simulink model "Pay_load"  (R2025a)
settings: Solver=ode4  StartTime=0.0  StopTime=1  FixedStep=0.001  RelTol=1e-3
values from neighbouring files (symbols this model uses):
  angle1_init = [0;0;0.3]    [param.m]
  angle2_init = [0;0;0.3]    [param.m]
  angle3_init = [0;0;0.3]    [param.m]
  angle4_init = [0;0;0.3]    [param.m]
  joint_matrix = [r1; r2; r3; r4]    [param.m]
  m1 = 1    [param.m]
  m2 = 1    [param.m]
  m3 = 1    [param.m]
  m4 = 1    [param.m]
  mL = 2    [param.m]
  P = block.DialogPrm(1).Data    [Load_dynamic.m]    (also in param.m = struct())
  p1_init = pL_init + RL_init*r1 - l1*e1    [param.m]
  p2_init = pL_init + RL_init*r2 - l2*e2    [param.m]
  p3_init = pL_init + RL_init*r3 - l3*e3    [param.m]
  p4_init = pL_init + RL_init*r4 - l4*e4    [param.m]
  r1 = [ 0.25; -0.20; -0.45]    [param.m]
  r2 = [-0.50; -0.40; -0.15]    [param.m]
  r3 = [-0.50;  0.40;  0.15]    [param.m]
  r4 = [ 0.50;  0.40;  0.00]    [param.m]
  xL_init = [pL_init; vL_init; angle_L_init; omega_L_init]    [param.m]
(part 1 of 3)
settings Model: Creator=huy01  LastModifiedBy=huy01

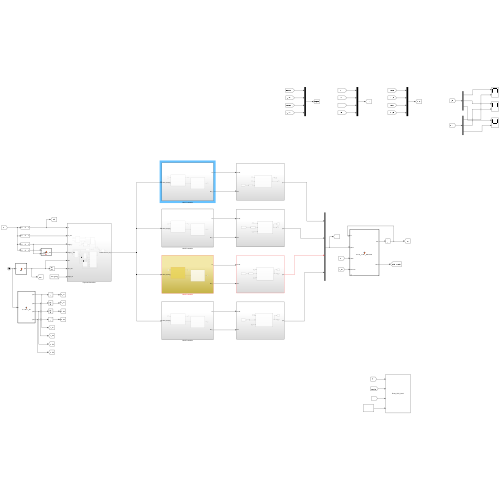
[thumbnail: Simulink's stored preview of the top-level diagram]
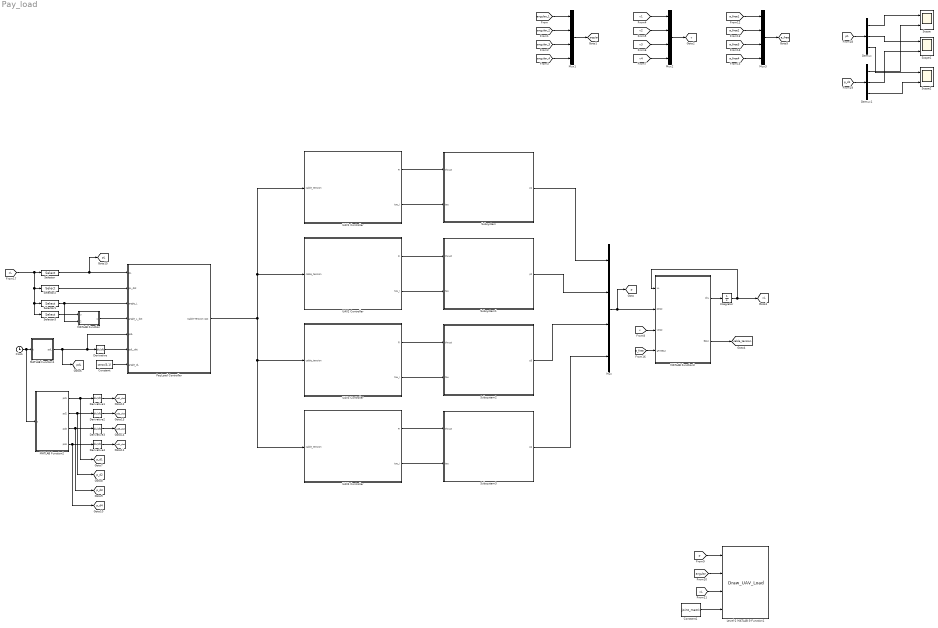
== system Pay_load ==
  Clock : Clock
  Constant : Constant  Value=zeros(3,1)
  Constant1 : Constant  Value=joint_matrix
  Demux : Demux  Outputs=3
  Demux1 : Demux  Outputs=3
  Derivative{,1..4} (5 alike) : Derivative
  Integrator : Integrator  InitialCondition=xL_init
  Level-2 MATLAB S-Function1 : M-S-Function  FunctionName=Draw_UAV_Load
  MATLAB Function : MATLAB Function  TreatAsAtomicUnit=on
  MATLAB Function1 : MATLAB Function  TreatAsAtomicUnit=on
  MATLAB Function2 : MATLAB Function  TreatAsAtomicUnit=on
  MATLAB Function3 : MATLAB Function  TreatAsAtomicUnit=on  mask{P=P}
      mask prompts: P "Struct param"
  Mux{,1..3} (4 alike) : Mux
  PayLoad Controller : Subsystem
  Scope : Scope  NumInputPorts=2
      settings: ActiveDisplayYMinimum=-0.075646367743774853  ActiveDisplayYMaximum=0.68476273102431728  DataLoggingVariableName=ScopeData15
  Scope1 : Scope  NumInputPorts=2
      settings: ActiveDisplayYMinimum=-1  ActiveDisplayYMaximum=1  DataLoggingVariableName=ScopeData16
  Scope2 : Scope  NumInputPorts=2
      settings: ActiveDisplayYMinimum=-13.522817048358654  ActiveDisplayYMaximum=4.0434204808418635  DataLoggingVariableName=ScopeData17
  Selector : Selector  InputPortWidth=12  IndexOptions=Index vector (dialog)  Indices=[1:3]  OutputSizes=1
  Selector1 : Selector  InputPortWidth=12  IndexOptions=Index vector (dialog)  Indices=[7:9]  OutputSizes=1
  Selector2 : Selector  InputPortWidth=12  IndexOptions=Index vector (dialog)  Indices=[4:6]  OutputSizes=1
  Selector3 : Selector  InputPortWidth=12  IndexOptions=Index vector (dialog)  Indices=[10:12]  OutputSizes=1
  Subsystem : Subsystem
  Subsystem1 : Subsystem
  Subsystem2 : Subsystem
  Subsystem3 : Subsystem
  UAV1 Controller : Subsystem
  UAV2 Controller : Subsystem
  UAV3 Controller : Subsystem
  UAV4 Controller : Subsystem
  tag scope: a_free=global, angular=global, cable_tension=global, p=global, pL=global, p_d1=global, p_d2=global, p_d3=global, p_d4=global, pd1_dot=global, pd2_dot=global, pd3_dot=global, pd4_dot=global, pdL=global, v=global, xL=global
  wires:
  Subsystem1/1(p2) -> Mux/2
  Subsystem2/1(p3) -> Mux/3
  Subsystem3/1(p4) -> Mux/4
  Subsystem/1(p1) -> Mux/1
  Mux/1 -> [p], MATLAB Function3/2(pD12)
  [angular_2] -> Mux1/2
  [angular_1] -> Mux1/1
  [angular_3] -> Mux1/3
  [angular_4] -> Mux1/4
  Mux1/1 -> [angular]
  [v4] -> Mux2/4
  [v3] -> Mux2/3
  [v1] -> Mux2/1
  Mux2/1 -> [v]
  [v2] -> Mux2/2
  [v] -> MATLAB Function3/3(vD12)
  Integrator/1 -> [xL], MATLAB Function3/1(xL)
  MATLAB Function3/2(fD12) -> [cable_tension]
  [p] -> Level-2 MATLAB S-Function1/1
  [angular] -> Level-2 MATLAB S-Function1/2
  [xL] -> Level-2 MATLAB S-Function1/3
  [a_free1] -> Mux3/1
  [a_free4] -> Mux3/4
  Mux3/1 -> [a_free]
  [a_free3] -> Mux3/3
  [a_free2] -> Mux3/2
  [a_free] -> MATLAB Function3/4(aFree12)
  Constant1/1 -> Level-2 MATLAB S-Function1/4
  Selector/1 -> [pL], PayLoad Controller/1(pL)
  [xL] -> Selector2/1, Selector1/1, Selector3/1, Selector/1
  Selector1/1 -> MATLAB Function/2(angle_L), PayLoad Controller/3(angle_L)
  Selector2/1 -> PayLoad Controller/2(pL_dot)
  UAV1 Controller/1(Fi) -> Subsystem/1(thrust)
  UAV1 Controller/2(tau_i) -> Subsystem/2(tau)
  UAV2 Controller/1(Fi) -> Subsystem1/1(thrust)
  UAV2 Controller/2(tau_i) -> Subsystem1/2(tau)
  UAV3 Controller/1(Fi) -> Subsystem2/1(thrust)
  UAV3 Controller/2(tau_i) -> Subsystem2/2(tau)
  UAV4 Controller/1(Fi) -> Subsystem3/1(thrust)
  UAV4 Controller/2(tau_i) -> Subsystem3/2(tau)
  PayLoad Controller/1(Cable Tension [12]) -> UAV2 Controller/1(cable_tension), UAV1 Controller/1(cable_tension), UAV4 Controller/1(cable_tension), UAV3 Controller/1(cable_tension)
  Selector3/1 -> MATLAB Function/1(u)
  MATLAB Function/1(angle_L_dot) -> PayLoad Controller/4(angle_L_dot)
  Clock/1 -> MATLAB Function2/1(t), MATLAB Function1/1(t)
  Derivative/1 -> PayLoad Controller/6(pdL_dot)
  Constant/1 -> PayLoad Controller/7(angle_dL)
  MATLAB Function1/1(pdL) -> [pdL], PayLoad Controller/5(pdL), Derivative/1
  MATLAB Function2/1(pd1) -> Derivative1/1, [p_d1]
  MATLAB Function2/2(pd2) -> Derivative2/1, [p_d2]
  MATLAB Function2/3(pd3) -> Derivative3/1, [p_d3]
  MATLAB Function2/4(pd4) -> Derivative4/1, [p_d4]
  Derivative1/1 -> [pd1_dot]
  Derivative2/1 -> [pd2_dot]
  Derivative3/1 -> [pd3_dot]
  Derivative4/1 -> [pd4_dot]
  MATLAB Function3/1(dxL) -> Integrator/1
  [p1] -> Demux/1
  [p_d1] -> Demux1/1
  Demux/1 -> Scope/1
  Demux1/1 -> Scope/2
  Demux/2 -> Scope1/1
  Demux1/2 -> Scope1/2
  Demux1/3 -> Scope2/2
  Demux/3 -> Scope2/1

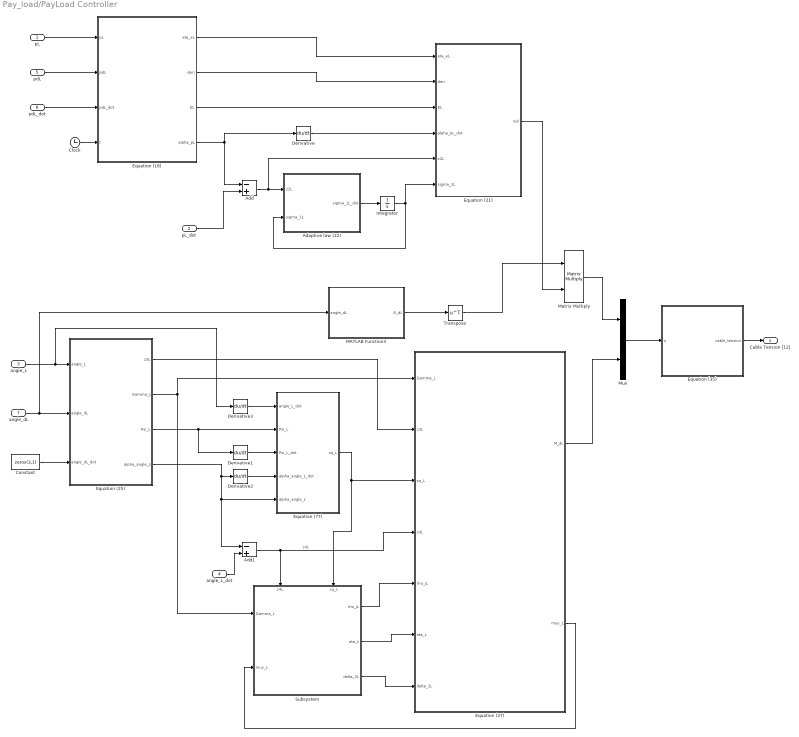
== system Pay_load/PayLoad Controller ==
  pL : Inport
  pL_dot : Inport  Port=2
  angle_L : Inport  Port=3
  angle_L_dot : Inport  Port=4
  pdL : Inport  Port=5
  pdL_dot : Inport  Port=6
  angle_dL : Inport  Port=7
  Adaptive law (22) : MATLAB Function  TreatAsAtomicUnit=on
  Add : Sum  Inputs=-+
  Add1 : Sum  Inputs=-+
  Clock : Clock
  Constant : Constant  Value=zeros(3,1)
  Derivative{,1..3} (4 alike) : Derivative
  Equation (18) : MATLAB Function  TreatAsAtomicUnit=on
  Equation (21) : MATLAB Function  TreatAsAtomicUnit=on  mask{Parameter1=mL}
      mask prompts: Parameter1 "Mass of Load"
  Equation (25) : MATLAB Function  TreatAsAtomicUnit=on
  Equation (27) : MATLAB Function  TreatAsAtomicUnit=on
  Equation (35) : MATLAB Function  TreatAsAtomicUnit=on  mask{joint_matrix=joint_matrix}
      mask prompts: joint_matrix "Joint Matrix"
  Equation (77) : MATLAB Function  TreatAsAtomicUnit=on
  Integrator : Integrator
  MATLAB Function3 : MATLAB Function  TreatAsAtomicUnit=on
  Matrix Multiply : Product  Multiplication=Matrix(*)
  Mux : Mux  Inputs=2
  Subsystem : Subsystem
      settings: PortSchema="{\"entries\":[{\"content\":{\"sides\":[{\"content\":{\"connectorIds\":[\"In1\",\"In2\"]},\"type\":\"ConnectorPlacement.EquallySpacedRectSide\",\"uuid\":\"85bb0074-8536-4f6f-9381-283f28dbadf4\"},{\"content\":{\"connectorIds\":[\"Out1\",\"Out2\",\"Out3\"],\"side\":\"RIGHT\"},\"type\":\"ConnectorPlacement.EquallySpacedRectSide\",\"uuid\":\"6437b79b-8dbf-4b76-9004-0601bc1c010e\"},{\"content\":{\"connectorIds\":[\"In3\",\"In4\"],\"side\":\"TOP\"},\"type\":\"ConnectorPlacement.EquallySpacedRectSide\",\"uuid\":\"271b864e-fd64-4648-b0f9-d789d7babcd4\"}]},\"type\":\"ConnectorPlacement.EquallySpacedConnector\",\"uuid\":\"6eb46f38-4b3a-4a47-bdc3-5643058b700a\"}],\"packageUris\":[\"http://schema.mathworks.com/mf0/Connector/R2020b\"],\"version\":\"1.0\"}"
  Transpose : Math  Operator=transpose
  Cable Tension [12] : Outport
  wires:
  pL/1 -> Equation (18)/1(pL)
  pdL/1 -> Equation (18)/2(pdL)
  pdL_dot/1 -> Equation (18)/3(pdL_dot)
  Clock/1 -> Equation (18)/4(t)
  Equation (18)/4(alpha_pL) -> Add/1, Derivative/1
  pL_dot/1 -> Add/2
  Adaptive law (22)/1(sigma_1L_dot) -> Integrator/1
  Integrator/1 -> Adaptive law (22)/2(sigma_1L), Equation (21)/6(sigma_1L)
  Add/1 -> Equation (21)/5(z2L), Adaptive law (22)/1(z2L)
  Derivative/1 -> Equation (21)/4(alpha_pL_dot)
  Equation (18)/3(EL) -> Equation (21)/3(EL)
  angle_L/1 -> Derivative3/1, Equation (25)/1(angle_L)
  angle_dL/1 -> MATLAB Function3/1(angle_dL), Equation (25)/2(angle_dL)
  angle_L_dot/1 -> Add1/2
  Add1/1 -> Equation (27)/4(z4L), Subsystem/3(z4L)  "z4L"
  Equation (25)/1(z3L) -> Equation (27)/2(z3L)
  Subsystem/1(rho_jL) -> Equation (27)/5(rho_jL)
  Subsystem/2(eta_L) -> Equation (27)/6(eta_L)
  Subsystem/3(delta_2L) -> Equation (27)/7(delta_2L)
  Equation (27)/2(muy_L) -> Subsystem/2(muy_L)
  MATLAB Function3/1(R_dL) -> Transpose/1
  Equation (21)/1(Fdl) -> Matrix Multiply/2
  Matrix Multiply/1 -> Mux/1
  Equation (27)/1(M_dL) -> Mux/2
  Transpose/1 -> Matrix Multiply/1
  Mux/1 -> Equation (35)/1(u)
  Equation (25)/2(Gamma_L) -> Subsystem/1(Gamma_L), Equation (27)/1(Gamma_L)
  Derivative1/1 -> Equation (77)/3(Psi_L_dot)
  Derivative2/1 -> Equation (77)/4(alpha_angle_L_dot)
  Equation (25)/4(alpha_angle_L) -> Add1/1, Equation (77)/5(alpha_angle_L), Derivative2/1
  Derivative3/1 -> Equation (77)/1(angle_L_dot)
  Equation (77)/1(sq_L) -> Equation (27)/3(sq_L), Subsystem/4(sq_L)
  Equation (35)/1(cable_tension) -> Cable Tension [12]/1
  Equation (25)/3(Psi_L) -> Derivative1/1, Equation (77)/2(Psi_L)
  Equation (18)/1(eta_eL) -> Equation (21)/1(eta_eL)
  Equation (18)/2(deri) -> Equation (21)/2(deri)
  Constant/1 -> Equation (25)/3(angle_dL_dot)

== system Pay_load/Subsystem ==
  thrust : Inport
  tau : Inport  Port=2
  Selector : Selector  InputPortWidth=12  IndexOptions=Index vector (dialog)  Indices=[1:3]  OutputSizes=1
  UAV1 : Subsystem
  p1 : Outport
  tag scope: p1=global
  wires:
  thrust/1 -> UAV1/1(thrust)
  UAV1/1(p1) -> [p1], p1/1
  tau/1 -> UAV1/2(tau)
  [cable_tension] -> Selector/1
  Selector/1 -> UAV1/3(cable_tension)

== system Pay_load/Subsystem1 ==
  thrust : Inport
  tau : Inport  Port=2
  Selector : Selector  InputPortWidth=12  IndexOptions=Index vector (dialog)  Indices=[4:6]  OutputSizes=1
  UAV2 : Subsystem
  p2 : Outport
  tag scope: p2=global
  wires:
  thrust/1 -> UAV2/1(thrust)
  UAV2/1(p2) -> [p2], p2/1
  tau/1 -> UAV2/3(tau)
  [cable_tension] -> Selector/1
  Selector/1 -> UAV2/2(cable_tension)

== system Pay_load/Subsystem2 ==
  thrust : Inport
  tau : Inport  Port=2
  Selector : Selector  InputPortWidth=12  IndexOptions=Index vector (dialog)  Indices=[7:9]  OutputSizes=1
  UAV3 : Subsystem
  p3 : Outport
  tag scope: p3=global
  wires:
  thrust/1 -> UAV3/1(thrust)
  tau/1 -> UAV3/3(tau)
  UAV3/1(p3) -> [p3], p3/1
  [cable_tension] -> Selector/1
  Selector/1 -> UAV3/2(cable_tension)

== system Pay_load/Subsystem3 ==
  thrust : Inport
  tau : Inport  Port=2
  Selector : Selector  InputPortWidth=12  IndexOptions=Index vector (dialog)  Indices=[10:12]  OutputSizes=1
  UAV4 : Subsystem
  p4 : Outport
  tag scope: p4=global
  wires:
  UAV4/1(p4) -> [p4], p4/1
  tau/1 -> UAV4/3(tau)
  thrust/1 -> UAV4/1(thrust)
  [cable_tension] -> Selector/1
  Selector/1 -> UAV4/2(cable_tension)

== system Pay_load/UAV1 Controller ==
  cable_tension : Inport
  Subsystem : Subsystem
  Subsystem1 : Subsystem
  Fi : Outport
  tau_i : Outport  Port=2
  wires:
  cable_tension/1 -> Subsystem1/2(cable_tension)
  Subsystem1/2(angle_di) -> Subsystem/1(angle_di)
  Subsystem1/1(Fi) -> Fi/1
  Subsystem/1(tau_i) -> tau_i/1
  [p_d1] -> Subsystem1/1(p_d1)

== system Pay_load/UAV2 Controller ==
  cable_tension : Inport
  Subsystem : Subsystem
  Subsystem1 : Subsystem
  Fi : Outport
  tau_i : Outport  Port=2
  wires:
  cable_tension/1 -> Subsystem1/2(cable_tension)
  Subsystem1/2(angle_di) -> Subsystem/1(angle_di)
  Subsystem1/1(Fi) -> Fi/1
  Subsystem/1(tau_i) -> tau_i/1
  [p_d2] -> Subsystem1/1(p_d1)

== system Pay_load/UAV3 Controller ==
  cable_tension : Inport
  Subsystem : Subsystem
  Subsystem1 : Subsystem
  Fi : Outport
  tau_i : Outport  Port=2
  wires:
  cable_tension/1 -> Subsystem1/2(cable_tension)
  Subsystem1/2(angle_di) -> Subsystem/1(angle_di)
  Subsystem1/1(Fi) -> Fi/1
  Subsystem/1(tau_i) -> tau_i/1
  [p_d3] -> Subsystem1/1(p_d1)

== system Pay_load/UAV4 Controller ==
  cable_tension : Inport
  Subsystem : Subsystem
  Subsystem1 : Subsystem
  Fi : Outport
  tau_i : Outport  Port=2
  wires:
  cable_tension/1 -> Subsystem1/2(cable_tension)
  Subsystem1/2(angle_di) -> Subsystem/1(angle_di)
  Subsystem1/1(Fi) -> Fi/1
  Subsystem/1(tau_i) -> tau_i/1
  [p_d4] -> Subsystem1/1(p_d4)

== system Pay_load/PayLoad Controller/Subsystem ==
  Gamma_L : Inport
  muy_L : Inport  Port=2
  z4L : Inport  Port=3
  sq_L : Inport  Port=4
  Adaptive Law (eq. 29) : MATLAB Function  TreatAsAtomicUnit=on
  Adaptive Law (eq. 30) : MATLAB Function  TreatAsAtomicUnit=on
  Adaptive Law (eq. 31) : MATLAB Function  TreatAsAtomicUnit=on
  Integrator1 : Integrator  InitialCondition=1
  Integrator2 : Integrator
  Integrator3 : Integrator
  rho_jL : Outport
  eta_L : Outport  Port=2
  delta_2L : Outport  Port=3
  wires:
  z4L/1 -> Adaptive Law (eq. 29)/1(z4L), Adaptive Law (eq. 31)/1(z4L), Adaptive Law (eq. 30)/1(z4L)
  Integrator2/1 -> eta_L/1, Adaptive Law (eq. 30)/2(eta_L)
  muy_L/1 -> Adaptive Law (eq. 29)/4(muy_L)
  Adaptive Law (eq. 29)/1(rho_jL_dot) -> Integrator1/1
  Adaptive Law (eq. 31)/1(delta_2L_dot) -> Integrator3/1
  Integrator1/1 -> rho_jL/1, Adaptive Law (eq. 29)/2(rho_jL)
  Adaptive Law (eq. 30)/1(eta_L_dot) -> Integrator2/1
  Gamma_L/1 -> Adaptive Law (eq. 29)/3(Gamma_L)
  Integrator3/1 -> delta_2L/1, Adaptive Law (eq. 31)/2(delta_2L)
  sq_L/1 -> Adaptive Law (eq. 30)/3(sq_L)

== system Pay_load/Subsystem/UAV1 ==
  thrust : Inport
  tau : Inport  Port=2
  cable_tension : Inport  Port=3
  Integrator : Integrator  InitialCondition=zeros(3,1)
  Integrator1 : Integrator  InitialCondition=p1_init
  Integrator2 : Integrator
  Integrator3 : Integrator  InitialCondition=angle1_init
  MATLAB Function : MATLAB Function  TreatAsAtomicUnit=on
  MATLAB Function1 : MATLAB Function  TreatAsAtomicUnit=on
  MATLAB Function2 : MATLAB Function  TreatAsAtomicUnit=on
  MATLAB Function3 : MATLAB Function  TreatAsAtomicUnit=on
  p1 : Outport
  tag scope: a_free1=global, angular_1=global, omega1=global, v1=global
  wires:
  MATLAB Function/1(p_ddot) -> Integrator/1
  Integrator/1 -> Integrator1/1, [v1]
  Integrator1/1 -> p1/1
  MATLAB Function1/1(omega_dot) -> Integrator2/1
  Integrator2/1 -> [omega1], MATLAB Function1/2(omega), MATLAB Function2/2(omega)
  Integrator3/1 -> [angular_1], MATLAB Function3/2(angular), MATLAB Function2/1(angle)
  thrust/1 -> MATLAB Function3/1(thrust)
  tau/1 -> MATLAB Function1/1(tau)
  MATLAB Function2/1(angle_dot) -> Integrator3/1
  MATLAB Function3/1(a_free) -> [a_free1], MATLAB Function/1(a_free)
  cable_tension/1 -> MATLAB Function/2(fCableWorld)

== system Pay_load/Subsystem1/UAV2 ==
  thrust : Inport
  cable_tension : Inport  Port=2
  tau : Inport  Port=3
  Integrator : Integrator
  Integrator1 : Integrator  InitialCondition=p2_init
  Integrator2 : Integrator
  Integrator3 : Integrator  InitialCondition=angle2_init
  MATLAB Function : MATLAB Function  TreatAsAtomicUnit=on
  MATLAB Function1 : MATLAB Function  TreatAsAtomicUnit=on
  MATLAB Function2 : MATLAB Function  TreatAsAtomicUnit=on
  MATLAB Function3 : MATLAB Function  TreatAsAtomicUnit=on
  p2 : Outport
  tag scope: a_free2=global, angular_2=global, omega2=global, v2=global
  wires:
  MATLAB Function/1(p_ddot) -> Integrator/1
  Integrator/1 -> [v2], Integrator1/1
  Integrator1/1 -> p2/1
  MATLAB Function3/1(a_free) -> [a_free2], MATLAB Function/1(a_free)
  MATLAB Function2/1(angle_dot) -> Integrator3/1
  Integrator2/1 -> [omega2], MATLAB Function1/2(omega), MATLAB Function2/2(omega)
  tau/1 -> MATLAB Function1/1(tau)
  MATLAB Function1/1(omega_dot) -> Integrator2/1
  thrust/1 -> MATLAB Function3/1(thrust)
  Integrator3/1 -> MATLAB Function3/2(angular), MATLAB Function2/1(angle), [angular_2]
  cable_tension/1 -> MATLAB Function/2(fCableWorld)

== system Pay_load/Subsystem2/UAV3 ==
  thrust : Inport
  cable_tension : Inport  Port=2
  tau : Inport  Port=3
  Integrator : Integrator
  Integrator1 : Integrator  InitialCondition=p3_init
  Integrator2 : Integrator
  Integrator3 : Integrator  InitialCondition=angle3_init
  MATLAB Function : MATLAB Function  TreatAsAtomicUnit=on
  MATLAB Function1 : MATLAB Function  TreatAsAtomicUnit=on
  MATLAB Function2 : MATLAB Function  TreatAsAtomicUnit=on
  MATLAB Function3 : MATLAB Function  TreatAsAtomicUnit=on
  p3 : Outport
  tag scope: a_free3=global, angular_3=global, omega3=global, v3=global
  wires:
  MATLAB Function/1(p_ddot) -> Integrator/1
  Integrator/1 -> [v3], Integrator1/1
  Integrator1/1 -> p3/1
  Integrator3/1 -> MATLAB Function2/1(angle), MATLAB Function3/2(angular), [angular_3]
  MATLAB Function3/1(a_free) -> [a_free3], MATLAB Function/1(a_free)
  MATLAB Function2/1(angle_dot) -> Integrator3/1
  Integrator2/1 -> [omega3], MATLAB Function1/2(omega), MATLAB Function2/2(omega)
  tau/1 -> MATLAB Function1/1(tau)
  MATLAB Function1/1(omega_dot) -> Integrator2/1
  thrust/1 -> MATLAB Function3/1(thrust)
  cable_tension/1 -> MATLAB Function/2(fCableWorld)

== system Pay_load/Subsystem3/UAV4 ==
  thrust : Inport
  cable_tension : Inport  Port=2
  tau : Inport  Port=3
  Integrator : Integrator
  Integrator1 : Integrator  InitialCondition=p4_init
  Integrator2 : Integrator  InitialCondition=zeros(3,1)
  Integrator3 : Integrator  InitialCondition=angle4_init
  MATLAB Function : MATLAB Function  TreatAsAtomicUnit=on
  MATLAB Function1 : MATLAB Function  TreatAsAtomicUnit=on
  MATLAB Function2 : MATLAB Function  TreatAsAtomicUnit=on
  MATLAB Function3 : MATLAB Function  TreatAsAtomicUnit=on
  p4 : Outport
  tag scope: a_free4=global, angular_4=global, omega4=global, v4=global
  wires:
  MATLAB Function/1(p_ddot) -> Integrator/1
  Integrator/1 -> [v4], Integrator1/1
  Integrator1/1 -> p4/1
  Integrator3/1 -> MATLAB Function3/2(angular), MATLAB Function2/1(angle), [angular_4]
  MATLAB Function3/1(a_free) -> [a_free4], MATLAB Function/1(a_free)
  MATLAB Function2/1(angle_dot) -> Integrator3/1
  Integrator2/1 -> [omega4], MATLAB Function1/2(omega), MATLAB Function2/2(omega)
  tau/1 -> MATLAB Function1/1(tau)
  MATLAB Function1/1(omega_dot) -> Integrator2/1
  thrust/1 -> MATLAB Function3/1(thrust)
  cable_tension/1 -> MATLAB Function/2(fCableWorld)

== system Pay_load/UAV1 Controller/Subsystem ==
  angle_di : Inport
  Integrator : Integrator  InitialCondition=1
  Integrator1 : Integrator
  MATLAB Function : MATLAB Function  TreatAsAtomicUnit=on
  MATLAB Function1 : MATLAB Function  TreatAsAtomicUnit=on
  MATLAB Function2 : MATLAB Function  TreatAsAtomicUnit=on
  Scope : Scope  NumInputPorts=2
  tau_i : Outport
  wires:
  [angular_1] -> MATLAB Function/1(angle_i)
  [omega1] -> MATLAB Function/2(omega_i)
  angle_di/1 -> MATLAB Function/3(angle_di)
  MATLAB Function/4(alpha_angle_i) -> MATLAB Function1/1(alpha_angle_i)
  MATLAB Function/5(angle_i_dot) -> MATLAB Function1/2(angle_i_dot)
  MATLAB Function/6(Psi_i) -> MATLAB Function2/4(Psi_i), MATLAB Function1/3(Psi_i)
  MATLAB Function/7(Psi_i_dot) -> MATLAB Function1/4(Psi_i_dot)
  MATLAB Function/1(z3i) -> Scope/1, MATLAB Function2/1(z3i)
  MATLAB Function/2(z4i) -> MATLAB Function2/2(z4i), Scope/2
  MATLAB Function/3(Gamma_i) -> MATLAB Function2/3(Gamma_i)
  MATLAB Function1/1(Xi_i) -> MATLAB Function2/5(Xi_i)
  MATLAB Function2/3(rho_Ji_dot) -> Integrator/1
  Integrator/1 -> MATLAB Function2/6(rho_Ji)
  MATLAB Function2/4(zeta_i_dot) -> Integrator1/1
  Integrator1/1 -> MATLAB Function2/7(zeta_i)
  MATLAB Function2/1(tau_i) -> tau_i/1

== system Pay_load/UAV1 Controller/Subsystem1 ==
  p_d1 : Inport
  cable_tension : Inport  Port=2
  Position Controller : Subsystem
  Subsystem : Subsystem
  Fi : Outport
  angle_di : Outport  Port=2
  wires:
  cable_tension/1 -> Subsystem/3(cable_tension)
  Position Controller/2(Ei) -> Subsystem/2(Ei)
  Position Controller/1(alpha_pi) -> Subsystem/1(alpha_pi)
  p_d1/1 -> Position Controller/1(p_d1)
  Subsystem/1(Fi) -> Fi/1
  Subsystem/2(angle_di) -> angle_di/1

== system Pay_load/UAV2 Controller/Subsystem ==
  angle_di : Inport
  Integrator : Integrator  InitialCondition=1
  Integrator1 : Integrator
  MATLAB Function : MATLAB Function  TreatAsAtomicUnit=on
  MATLAB Function1 : MATLAB Function  TreatAsAtomicUnit=on
  MATLAB Function2 : MATLAB Function  TreatAsAtomicUnit=on
  Scope : Scope  NumInputPorts=2
  tau_i : Outport
  wires:
  [angular_2] -> MATLAB Function/1(angle_i)
  [omega2] -> MATLAB Function/2(omega_i)
  angle_di/1 -> MATLAB Function/3(angle_di)
  MATLAB Function/4(alpha_angle_i) -> MATLAB Function1/1(alpha_angle_i)
  MATLAB Function/5(angle_i_dot) -> MATLAB Function1/2(angle_i_dot)
  MATLAB Function/6(Psi_i) -> MATLAB Function2/4(Psi_i), MATLAB Function1/3(Psi_i)
  MATLAB Function/7(Psi_i_dot) -> MATLAB Function1/4(Psi_i_dot)
  MATLAB Function/1(z3i) -> Scope/1, MATLAB Function2/1(z3i)
  MATLAB Function/2(z4i) -> MATLAB Function2/2(z4i), Scope/2
  MATLAB Function/3(Gamma_i) -> MATLAB Function2/3(Gamma_i)
  MATLAB Function1/1(Xi_i) -> MATLAB Function2/5(Xi_i)
  MATLAB Function2/3(rho_Ji_dot) -> Integrator/1
  Integrator/1 -> MATLAB Function2/6(rho_Ji)
  MATLAB Function2/4(zeta_i_dot) -> Integrator1/1
  Integrator1/1 -> MATLAB Function2/7(zeta_i)
  MATLAB Function2/1(tau_i) -> tau_i/1

== system Pay_load/UAV2 Controller/Subsystem1 ==
  p_d1 : Inport
  cable_tension : Inport  Port=2
  Position Controller : Subsystem
  Subsystem : Subsystem
  Fi : Outport
  angle_di : Outport  Port=2
  wires:
  cable_tension/1 -> Subsystem/3(cable_tension)
  Position Controller/2(Ei) -> Subsystem/2(Ei)
  Position Controller/1(alpha_pi) -> Subsystem/1(alpha_pi)
  p_d1/1 -> Position Controller/1(p_d2)
  Subsystem/1(Fi) -> Fi/1
  Subsystem/2(angle_di) -> angle_di/1

== system Pay_load/UAV3 Controller/Subsystem ==
  angle_di : Inport
  Integrator : Integrator  InitialCondition=1
  Integrator1 : Integrator
  MATLAB Function : MATLAB Function  TreatAsAtomicUnit=on
  MATLAB Function1 : MATLAB Function  TreatAsAtomicUnit=on
  MATLAB Function2 : MATLAB Function  TreatAsAtomicUnit=on
  Scope : Scope  NumInputPorts=2
  tau_i : Outport
  wires:
  [angular_3] -> MATLAB Function/1(angle_i)
  [omega3] -> MATLAB Function/2(omega_i)
  angle_di/1 -> MATLAB Function/3(angle_di)
  MATLAB Function/4(alpha_angle_i) -> MATLAB Function1/1(alpha_angle_i)
  MATLAB Function/5(angle_i_dot) -> MATLAB Function1/2(angle_i_dot)
  MATLAB Function/6(Psi_i) -> MATLAB Function2/4(Psi_i), MATLAB Function1/3(Psi_i)
  MATLAB Function/7(Psi_i_dot) -> MATLAB Function1/4(Psi_i_dot)
  MATLAB Function/1(z3i) -> Scope/1, MATLAB Function2/1(z3i)
  MATLAB Function/2(z4i) -> MATLAB Function2/2(z4i), Scope/2
  MATLAB Function/3(Gamma_i) -> MATLAB Function2/3(Gamma_i)
  MATLAB Function1/1(Xi_i) -> MATLAB Function2/5(Xi_i)
  MATLAB Function2/3(rho_Ji_dot) -> Integrator/1
  Integrator/1 -> MATLAB Function2/6(rho_Ji)
  MATLAB Function2/4(zeta_i_dot) -> Integrator1/1
  Integrator1/1 -> MATLAB Function2/7(zeta_i)
  MATLAB Function2/1(tau_i) -> tau_i/1

== system Pay_load/UAV3 Controller/Subsystem1 ==
  p_d1 : Inport
  cable_tension : Inport  Port=2
  Position Controller : Subsystem
  Subsystem : Subsystem
  Fi : Outport
  angle_di : Outport  Port=2
  wires:
  cable_tension/1 -> Subsystem/3(cable_tension)
  Position Controller/2(Ei) -> Subsystem/2(Ei)
  Position Controller/1(alpha_pi) -> Subsystem/1(alpha_pi)
  p_d1/1 -> Position Controller/1(p_d3)
  Subsystem/1(Fi) -> Fi/1
  Subsystem/2(angle_di) -> angle_di/1

== system Pay_load/UAV4 Controller/Subsystem ==
  angle_di : Inport
  Integrator : Integrator  InitialCondition=1
  Integrator1 : Integrator
  MATLAB Function : MATLAB Function  TreatAsAtomicUnit=on
  MATLAB Function1 : MATLAB Function  TreatAsAtomicUnit=on
  MATLAB Function2 : MATLAB Function  TreatAsAtomicUnit=on
  Scope : Scope  NumInputPorts=2
  tau_i : Outport
  wires:
  [angular_4] -> MATLAB Function/1(angle_i)
  [omega4] -> MATLAB Function/2(omega_i)
  angle_di/1 -> MATLAB Function/3(angle_di)
  MATLAB Function/4(alpha_angle_i) -> MATLAB Function1/1(alpha_angle_i)
  MATLAB Function/5(angle_i_dot) -> MATLAB Function1/2(angle_i_dot)
  MATLAB Function/6(Psi_i) -> MATLAB Function2/4(Psi_i), MATLAB Function1/3(Psi_i)
  MATLAB Function/7(Psi_i_dot) -> MATLAB Function1/4(Psi_i_dot)
  MATLAB Function/1(z3i) -> Scope/1, MATLAB Function2/1(z3i)
  MATLAB Function/2(z4i) -> MATLAB Function2/2(z4i), Scope/2
  MATLAB Function/3(Gamma_i) -> MATLAB Function2/3(Gamma_i)
  MATLAB Function1/1(Xi_i) -> MATLAB Function2/5(Xi_i)
  MATLAB Function2/3(rho_Ji_dot) -> Integrator/1
  Integrator/1 -> MATLAB Function2/6(rho_Ji)
  MATLAB Function2/4(zeta_i_dot) -> Integrator1/1
  Integrator1/1 -> MATLAB Function2/7(zeta_i)
  MATLAB Function2/1(tau_i) -> tau_i/1

== system Pay_load/UAV4 Controller/Subsystem1 ==
  p_d4 : Inport
  cable_tension : Inport  Port=2
  Position Controller : Subsystem
  Subsystem : Subsystem
  Fi : Outport
  angle_di : Outport  Port=2
  wires:
  cable_tension/1 -> Subsystem/3(cable_tension)
  Position Controller/2(Ei) -> Subsystem/2(Ei)
  Position Controller/1(alpha_pi) -> Subsystem/1(alpha_pi)
  p_d4/1 -> Position Controller/1(p_d4)
  Subsystem/1(Fi) -> Fi/1
  Subsystem/2(angle_di) -> angle_di/1

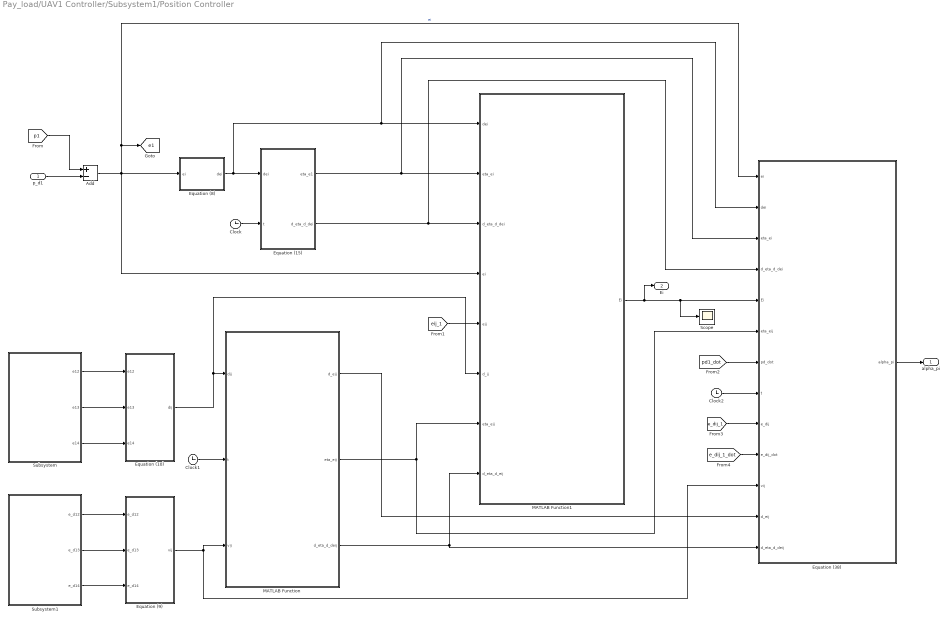
== system Pay_load/UAV1 Controller/Subsystem1/Position Controller ==
  p_d1 : Inport
  Add : Sum  Inputs=+-
  Clock : Clock
  Clock1 : Clock
  Clock2 : Clock
  Equation (10) : MATLAB Function  TreatAsAtomicUnit=on
  Equation (15) : MATLAB Function  TreatAsAtomicUnit=on
  Equation (38) : MATLAB Function  TreatAsAtomicUnit=on
  Equation (8) : MATLAB Function  TreatAsAtomicUnit=on
  Equation (9) : MATLAB Function  TreatAsAtomicUnit=on
  MATLAB Function : MATLAB Function  TreatAsAtomicUnit=on
  MATLAB Function1 : MATLAB Function  TreatAsAtomicUnit=on
  Scope : Scope
      settings: ActiveDisplayYMinimum=-1  ActiveDisplayYMaximum=1  DataLoggingVariableName=ScopeData4
  Subsystem : Subsystem
  Subsystem1 : Subsystem
  alpha_pi : Outport
  Ei : Outport  Port=2
  tag scope: e1=global
  wires:
  Subsystem1/1(e_d12) -> Equation (9)/1(e_d12)
  Equation (38)/1(alpha_pi) -> alpha_pi/1
  [e_dij_1_dot] -> Equation (38)/10(e_dij_dot)
  [pd1_dot] -> Equation (38)/7(pd_dot)
  MATLAB Function1/1(Ei) -> Ei/1, Scope/1, Equation (38)/5(Ei)
  [eij_1] -> MATLAB Function1/5(eij)
  Equation (15)/1(eta_e1) -> MATLAB Function1/2(eta_ei), Equation (38)/3(eta_ei)
  MATLAB Function/2(eta_eij) -> Equation (38)/6(eta_eij), MATLAB Function1/7(eta_eij)
  Equation (15)/2(d_eta_d_dei) -> MATLAB Function1/3(d_eta_d_dei), Equation (38)/4(d_eta_d_dei)
  Subsystem1/2(e_d13) -> Equation (9)/2(e_d13)
  MATLAB Function/1(d_eij) -> Equation (38)/12(d_eij)
  Subsystem/1(e12) -> Equation (10)/1(e12)
  Subsystem/3(e14) -> Equation (10)/3(e14)
  Clock1/1 -> MATLAB Function/2(t)
  MATLAB Function/3(d_eta_d_deij) -> Equation (38)/13(d_eta_d_deij), MATLAB Function1/8(d_eta_d_eij)
  [e_dij_1] -> Equation (38)/9(e_dij)
  p_d1/1 -> Add/2
  Clock/1 -> Equation (15)/2(t)
  Equation (9)/1(vij) -> Equation (38)/11(vij), MATLAB Function/3(vij)
  Equation (8)/1(dei) -> MATLAB Function1/1(dei), Equation (38)/2(dei), Equation (15)/1(dei)
  Subsystem/2(e13) -> Equation (10)/2(e13)
  [p1] -> Add/1
  Add/1 -> MATLAB Function1/4(ei), [e1], Equation (38)/1(ei), Equation (8)/1(ei)  "ei"
  Clock2/1 -> Equation (38)/8(t)
  Subsystem1/3(e_d14) -> Equation (9)/3(e_d14)
  Equation (10)/1(dij) -> MATLAB Function/1(dij), MATLAB Function1/6(d_ij)

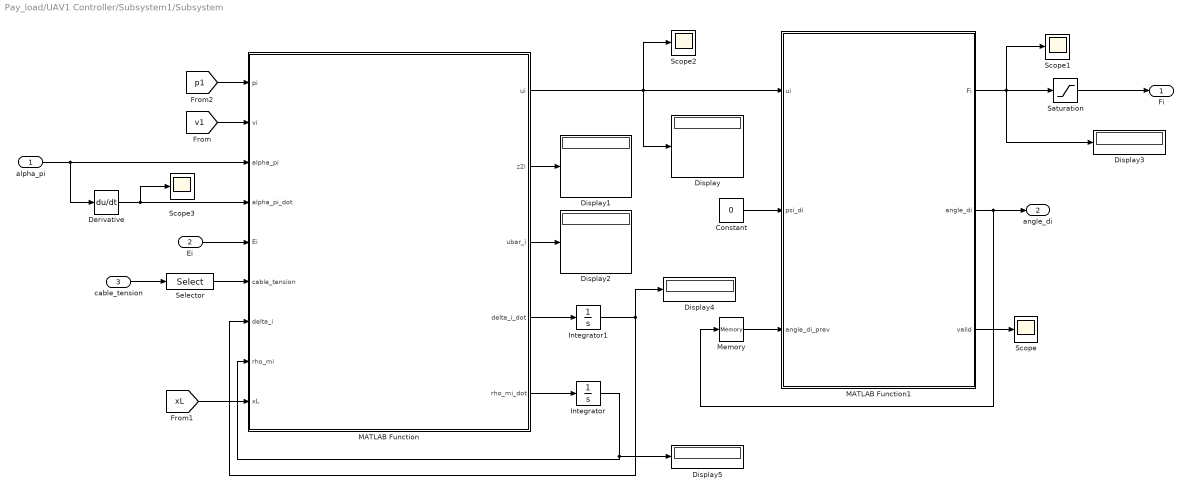
== system Pay_load/UAV1 Controller/Subsystem1/Subsystem ==
  alpha_pi : Inport
  Ei : Inport  Port=2
  cable_tension : Inport  Port=3
  Constant : Constant  Value=0
  Derivative : Derivative
  Display{,1..5} (6 alike) : Display
  Integrator : Integrator  InitialCondition=1
  Integrator1 : Integrator  InitialCondition=0.1
  MATLAB Function : MATLAB Function  TreatAsAtomicUnit=on  mask{ri=r1, m=m1}
      mask prompts: ri "Joint Vector"; m "UAV's Mass"
  MATLAB Function1 : MATLAB Function  TreatAsAtomicUnit=on
  Memory : Memory  InitialCondition=zeros(3,1)
  Saturation : Saturate  UpperLimit=75  LowerLimit=0
  Scope{,1..3} (4 alike) : Scope
      Scope1 settings: ActiveDisplayYMinimum=-1  ActiveDisplayYMaximum=1  DataLoggingVariableName=ScopeData2
      Scope2 settings: ActiveDisplayYMinimum=-15257.060994479718  ActiveDisplayYMaximum=31426.705160841346  DataLoggingVariableName=ScopeData3
      Scope3 settings: ActiveDisplayYMinimum=-1  ActiveDisplayYMaximum=1  DataLoggingVariableName=ScopeData5
  Selector : Selector  InputPortWidth=12  IndexOptions=Index vector (dialog)  Indices=[1:3]  OutputSizes=1
  Fi : Outport
  angle_di : Outport  Port=2
  wires:
  [v1] -> MATLAB Function/2(vi)
  alpha_pi/1 -> Derivative/1, MATLAB Function/3(alpha_pi)
  Ei/1 -> MATLAB Function/5(Ei)
  Derivative/1 -> Scope3/1, MATLAB Function/4(alpha_pi_dot)
  MATLAB Function/5(rho_mi_dot) -> Integrator/1
  MATLAB Function/4(delta_i_dot) -> Integrator1/1
  Integrator1/1 -> MATLAB Function/7(delta_i), Display4/1
  Integrator/1 -> MATLAB Function/8(rho_mi), Display5/1
  cable_tension/1 -> Selector/1
  Selector/1 -> MATLAB Function/6(cable_tension)
  [xL] -> MATLAB Function/9(xL)
  [p1] -> MATLAB Function/1(pi)
  MATLAB Function/1(ui) -> Display/1, Scope2/1, MATLAB Function1/1(ui)
  Constant/1 -> MATLAB Function1/2(psi_di)
  Memory/1 -> MATLAB Function1/3(angle_di_prev)
  MATLAB Function1/2(angle_di) -> angle_di/1, Memory/1
  MATLAB Function1/3(valid) -> Scope/1
  MATLAB Function1/1(Fi) -> Display3/1, Saturation/1, Scope1/1
  MATLAB Function/2(z2i) -> Display1/1
  MATLAB Function/3(ubar_i) -> Display2/1
  Saturation/1 -> Fi/1

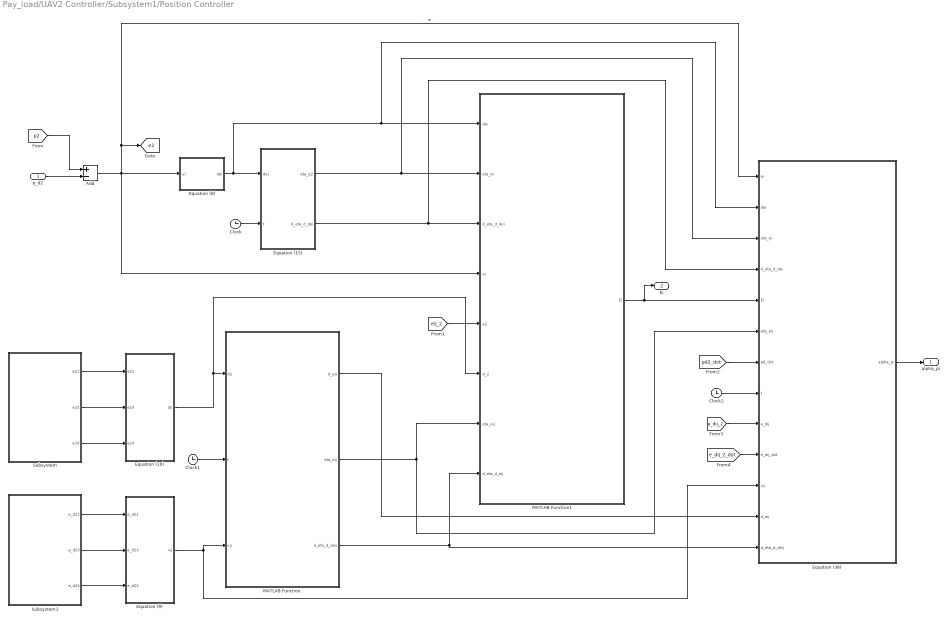
== system Pay_load/UAV2 Controller/Subsystem1/Position Controller ==
  p_d2 : Inport
  Add : Sum  Inputs=+-
  Clock : Clock
  Clock1 : Clock
  Clock2 : Clock
  Equation (10) : MATLAB Function  TreatAsAtomicUnit=on
  Equation (15) : MATLAB Function  TreatAsAtomicUnit=on
  Equation (38) : MATLAB Function  TreatAsAtomicUnit=on
  Equation (8) : MATLAB Function  TreatAsAtomicUnit=on
  Equation (9) : MATLAB Function  TreatAsAtomicUnit=on
  MATLAB Function : MATLAB Function  TreatAsAtomicUnit=on
  MATLAB Function1 : MATLAB Function  TreatAsAtomicUnit=on
  Subsystem : Subsystem
  Subsystem1 : Subsystem
  alpha_pi : Outport
  Ei : Outport  Port=2
  tag scope: e2=global
  wires:
  Subsystem1/1(e_d21) -> Equation (9)/1(e_d21)
  Equation (38)/1(alpha_pi) -> alpha_pi/1
  [e_dij_2_dot] -> Equation (38)/10(e_dij_dot)
  [pd2_dot] -> Equation (38)/7(pd_dot)
  MATLAB Function1/1(Ei) -> Ei/1, Equation (38)/5(Ei)
  [eij_2] -> MATLAB Function1/5(eij)
  Equation (15)/1(eta_e2) -> MATLAB Function1/2(eta_ei), Equation (38)/3(eta_ei)
  MATLAB Function/2(eta_eij) -> Equation (38)/6(eta_eij), MATLAB Function1/7(eta_eij)
  Equation (15)/2(d_eta_d_dei) -> MATLAB Function1/3(d_eta_d_dei), Equation (38)/4(d_eta_d_dei)
  Subsystem1/2(e_d23) -> Equation (9)/2(e_d23)
  MATLAB Function/1(d_eij) -> Equation (38)/12(d_eij)
  Subsystem/1(e21) -> Equation (10)/1(e21)
  Subsystem/3(e24) -> Equation (10)/3(e24)
  Clock1/1 -> MATLAB Function/2(t)
  MATLAB Function/3(d_eta_d_deij) -> Equation (38)/13(d_eta_d_deij), MATLAB Function1/8(d_eta_d_eij)
  [e_dij_2] -> Equation (38)/9(e_dij)
  p_d2/1 -> Add/2
  Clock/1 -> Equation (15)/2(t)
  Equation (9)/1(vij) -> Equation (38)/11(vij), MATLAB Function/3(vij)
  Equation (8)/1(dei) -> MATLAB Function1/1(dei), Equation (38)/2(dei), Equation (15)/1(dei)
  Subsystem/2(e23) -> Equation (10)/2(e23)
  [p2] -> Add/1
  Add/1 -> MATLAB Function1/4(ei), [e2], Equation (38)/1(ei), Equation (8)/1(ei)  "ei"
  Clock2/1 -> Equation (38)/8(t)
  Subsystem1/3(e_d24) -> Equation (9)/3(e_d24)
  Equation (10)/1(dij) -> MATLAB Function/1(dij), MATLAB Function1/6(d_ij)

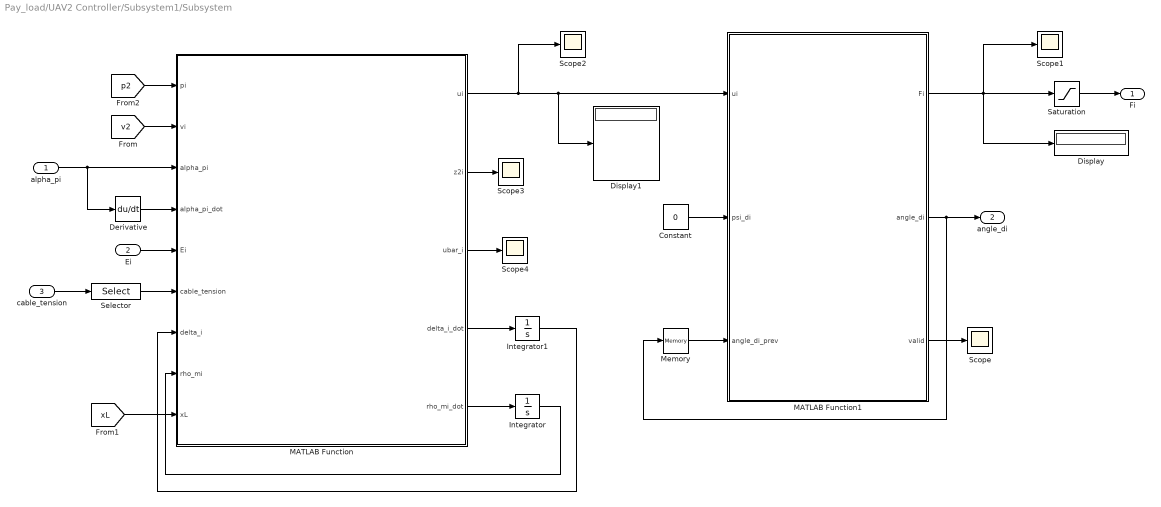
== system Pay_load/UAV2 Controller/Subsystem1/Subsystem ==
  alpha_pi : Inport
  Ei : Inport  Port=2
  cable_tension : Inport  Port=3
  Constant : Constant  Value=0
  Derivative : Derivative
  Display : Display
  Display1 : Display
  Integrator : Integrator  InitialCondition=1
  Integrator1 : Integrator
  MATLAB Function : MATLAB Function  TreatAsAtomicUnit=on  mask{ri=r2, m=m2}
      mask prompts: ri "Joint Vector"; m "UAV's Mass"
  MATLAB Function1 : MATLAB Function  TreatAsAtomicUnit=on
  Memory : Memory
  Saturation : Saturate  UpperLimit=75  LowerLimit=0
  Scope{,1..4} (5 alike) : Scope
      Scope1 settings: ActiveDisplayYMinimum=-1  ActiveDisplayYMaximum=1  DataLoggingVariableName=ScopeData10
      Scope2 settings: ActiveDisplayYMinimum=-1  ActiveDisplayYMaximum=1  DataLoggingVariableName=ScopeData11
      Scope3 settings: DataLoggingVariableName=ScopeData12
      Scope4 settings: DataLoggingVariableName=ScopeData13
  Selector : Selector  InputPortWidth=12  IndexOptions=Index vector (dialog)  Indices=[4:6]  OutputSizes=1
  Fi : Outport
  angle_di : Outport  Port=2
  wires:
  [v2] -> MATLAB Function/2(vi)
  alpha_pi/1 -> Derivative/1, MATLAB Function/3(alpha_pi)
  Ei/1 -> MATLAB Function/5(Ei)
  Derivative/1 -> MATLAB Function/4(alpha_pi_dot)
  MATLAB Function/5(rho_mi_dot) -> Integrator/1
  MATLAB Function/4(delta_i_dot) -> Integrator1/1
  Integrator1/1 -> MATLAB Function/7(delta_i)
  Integrator/1 -> MATLAB Function/8(rho_mi)
  cable_tension/1 -> Selector/1
  Selector/1 -> MATLAB Function/6(cable_tension)
  [xL] -> MATLAB Function/9(xL)
  [p2] -> MATLAB Function/1(pi)
  MATLAB Function/1(ui) -> Display1/1, MATLAB Function1/1(ui), Scope2/1
  Constant/1 -> MATLAB Function1/2(psi_di)
  Memory/1 -> MATLAB Function1/3(angle_di_prev)
  MATLAB Function1/2(angle_di) -> angle_di/1, Memory/1
  MATLAB Function1/3(valid) -> Scope/1
  MATLAB Function1/1(Fi) -> Display/1, Scope1/1, Saturation/1
  Saturation/1 -> Fi/1
  MATLAB Function/2(z2i) -> Scope3/1
  MATLAB Function/3(ubar_i) -> Scope4/1

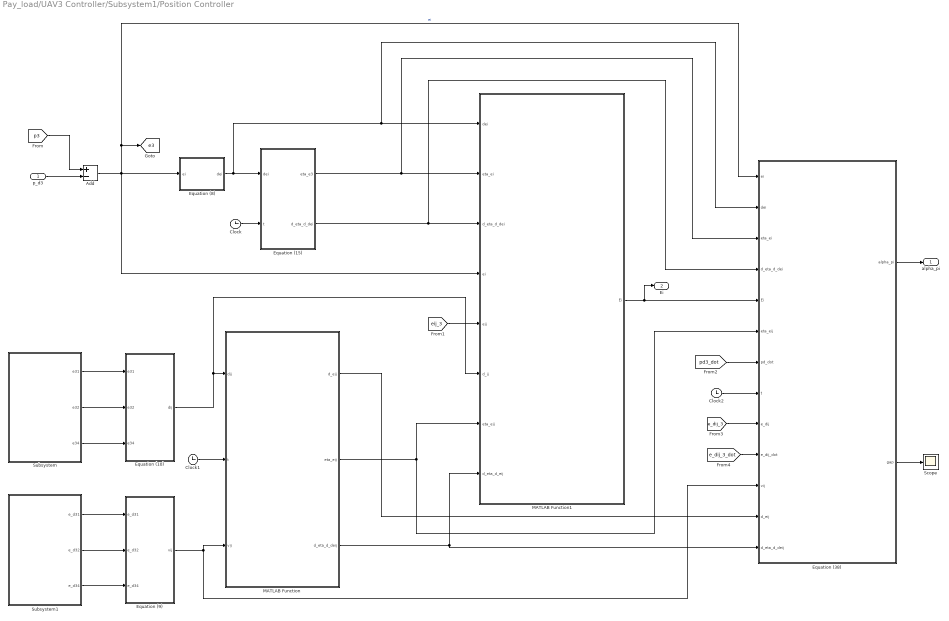
== system Pay_load/UAV3 Controller/Subsystem1/Position Controller ==
  p_d3 : Inport
  Add : Sum  Inputs=+-
  Clock : Clock
  Clock1 : Clock
  Clock2 : Clock
  Equation (10) : MATLAB Function  TreatAsAtomicUnit=on
  Equation (15) : MATLAB Function  TreatAsAtomicUnit=on
  Equation (38) : MATLAB Function  TreatAsAtomicUnit=on
  Equation (8) : MATLAB Function  TreatAsAtomicUnit=on
  Equation (9) : MATLAB Function  TreatAsAtomicUnit=on
  MATLAB Function : MATLAB Function  TreatAsAtomicUnit=on
  MATLAB Function1 : MATLAB Function  TreatAsAtomicUnit=on
  Scope : Scope
      settings: ActiveDisplayYMinimum=-1.785149854376475  ActiveDisplayYMaximum=7.088648176369837  DataLoggingVariableName=ScopeData22
  Subsystem : Subsystem
  Subsystem1 : Subsystem
  alpha_pi : Outport
  Ei : Outport  Port=2
  tag scope: e3=global
  wires:
  Subsystem1/1(e_d31) -> Equation (9)/1(e_d31)
  Equation (38)/1(alpha_pi) -> alpha_pi/1
  [e_dij_3_dot] -> Equation (38)/10(e_dij_dot)
  [pd3_dot] -> Equation (38)/7(pd_dot)
  MATLAB Function1/1(Ei) -> Ei/1, Equation (38)/5(Ei)
  [eij_3] -> MATLAB Function1/5(eij)
  Equation (15)/1(eta_e3) -> MATLAB Function1/2(eta_ei), Equation (38)/3(eta_ei)
  MATLAB Function/2(eta_eij) -> Equation (38)/6(eta_eij), MATLAB Function1/7(eta_eij)
  Equation (15)/2(d_eta_d_dei) -> MATLAB Function1/3(d_eta_d_dei), Equation (38)/4(d_eta_d_dei)
  Subsystem1/2(e_d32) -> Equation (9)/2(e_d32)
  MATLAB Function/1(d_eij) -> Equation (38)/12(d_eij)
  Subsystem/1(e31) -> Equation (10)/1(e31)
  Subsystem/3(e34) -> Equation (10)/3(e34)
  Clock1/1 -> MATLAB Function/2(t)
  MATLAB Function/3(d_eta_d_deij) -> Equation (38)/13(d_eta_d_deij), MATLAB Function1/8(d_eta_d_eij)
  [e_dij_3] -> Equation (38)/9(e_dij)
  p_d3/1 -> Add/2
  Clock/1 -> Equation (15)/2(t)
  Equation (9)/1(vij) -> Equation (38)/11(vij), MATLAB Function/3(vij)
  Equation (8)/1(dei) -> MATLAB Function1/1(dei), Equation (38)/2(dei), Equation (15)/1(dei)
  Subsystem/2(e32) -> Equation (10)/2(e32)
  [p3] -> Add/1
  Add/1 -> MATLAB Function1/4(ei), [e3], Equation (38)/1(ei), Equation (8)/1(ei)  "ei"
  Clock2/1 -> Equation (38)/8(t)
  Subsystem1/3(e_d34) -> Equation (9)/3(e_d34)
  Equation (10)/1(dij) -> MATLAB Function/1(dij), MATLAB Function1/6(d_ij)
  Equation (38)/2(gap) -> Scope/1

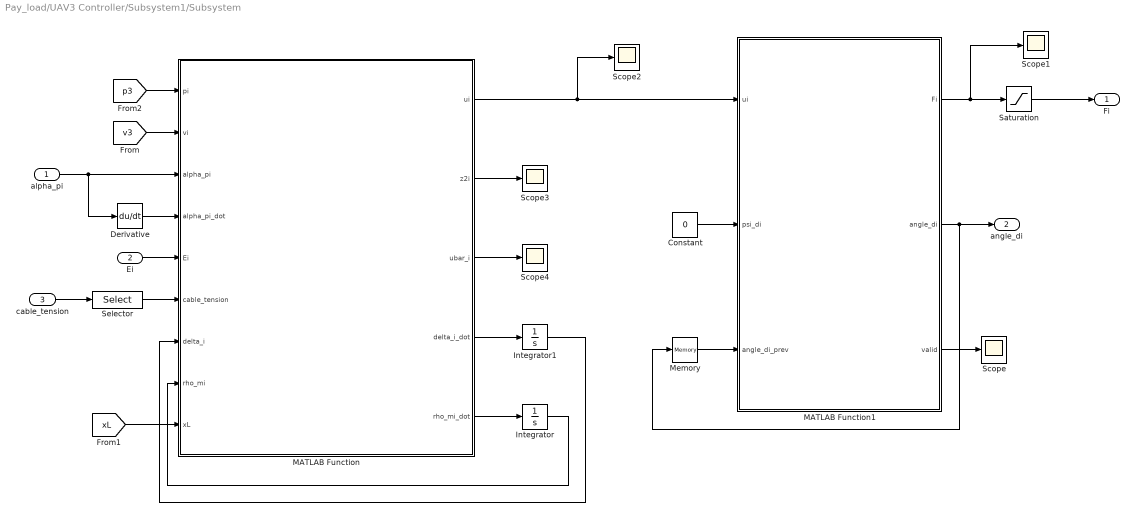
== system Pay_load/UAV3 Controller/Subsystem1/Subsystem ==
  alpha_pi : Inport
  Ei : Inport  Port=2
  cable_tension : Inport  Port=3
  Constant : Constant  Value=0
  Derivative : Derivative
  Integrator : Integrator  InitialCondition=1
  Integrator1 : Integrator
  MATLAB Function : MATLAB Function  TreatAsAtomicUnit=on  mask{ri=r3, m=m3}
      mask prompts: ri "Joint Vector"; m "UAV's Mass"
  MATLAB Function1 : MATLAB Function  TreatAsAtomicUnit=on
  Memory : Memory
  Saturation : Saturate  UpperLimit=75  LowerLimit=0
  Scope{,1..4} (5 alike) : Scope
      Scope1 settings: DataLoggingVariableName=ScopeData18
      Scope2 settings: ActiveDisplayYMinimum=-1.1356015539836052E+12  ActiveDisplayYMaximum=1.894440642846445E+11  DataLoggingVariableName=ScopeData19
      Scope3 settings: DataLoggingVariableName=ScopeData20
      Scope4 settings: DataLoggingVariableName=ScopeData21
  Selector : Selector  InputPortWidth=12  IndexOptions=Index vector (dialog)  Indices=[7:9]  OutputSizes=1
  Fi : Outport
  angle_di : Outport  Port=2
  wires:
  [v3] -> MATLAB Function/2(vi)
  alpha_pi/1 -> Derivative/1, MATLAB Function/3(alpha_pi)
  Ei/1 -> MATLAB Function/5(Ei)
  Derivative/1 -> MATLAB Function/4(alpha_pi_dot)
  MATLAB Function/5(rho_mi_dot) -> Integrator/1
  MATLAB Function/4(delta_i_dot) -> Integrator1/1
  Integrator1/1 -> MATLAB Function/7(delta_i)
  Integrator/1 -> MATLAB Function/8(rho_mi)
  cable_tension/1 -> Selector/1
  Selector/1 -> MATLAB Function/6(cable_tension)
  [xL] -> MATLAB Function/9(xL)
  [p3] -> MATLAB Function/1(pi)
  MATLAB Function/1(ui) -> Scope2/1, MATLAB Function1/1(ui)
  Constant/1 -> MATLAB Function1/2(psi_di)
  Memory/1 -> MATLAB Function1/3(angle_di_prev)
  MATLAB Function1/2(angle_di) -> angle_di/1, Memory/1
  MATLAB Function1/3(valid) -> Scope/1
  MATLAB Function1/1(Fi) -> Scope1/1, Saturation/1
  Saturation/1 -> Fi/1
  MATLAB Function/2(z2i) -> Scope3/1
  MATLAB Function/3(ubar_i) -> Scope4/1

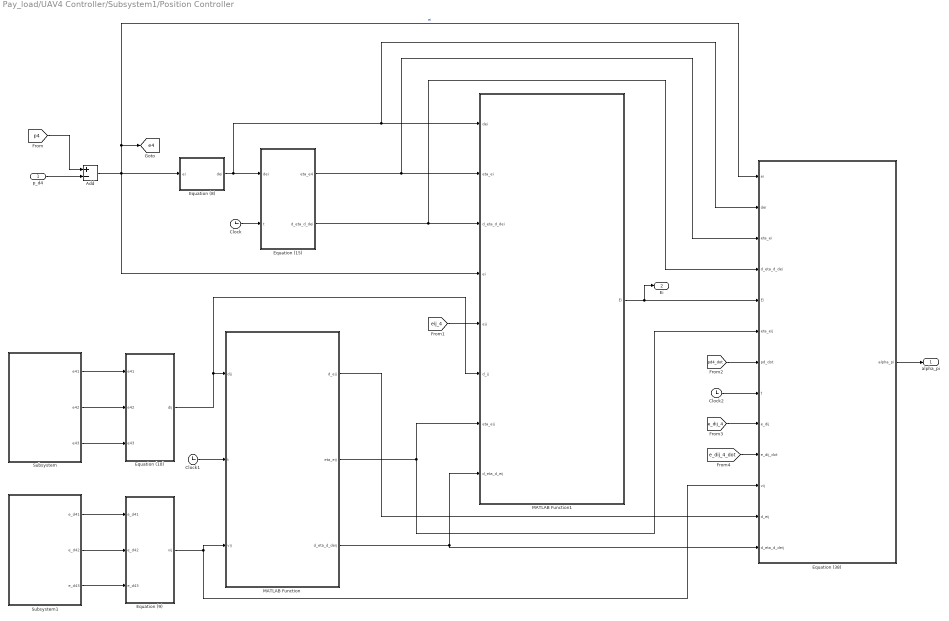
== system Pay_load/UAV4 Controller/Subsystem1/Position Controller ==
  p_d4 : Inport
  Add : Sum  Inputs=+-
  Clock : Clock
  Clock1 : Clock
  Clock2 : Clock
  Equation (10) : MATLAB Function  TreatAsAtomicUnit=on
  Equation (15) : MATLAB Function  TreatAsAtomicUnit=on
  Equation (38) : MATLAB Function  TreatAsAtomicUnit=on
  Equation (8) : MATLAB Function  TreatAsAtomicUnit=on
  Equation (9) : MATLAB Function  TreatAsAtomicUnit=on
  MATLAB Function : MATLAB Function  TreatAsAtomicUnit=on
  MATLAB Function1 : MATLAB Function  TreatAsAtomicUnit=on
  Subsystem : Subsystem
  Subsystem1 : Subsystem
  alpha_pi : Outport
  Ei : Outport  Port=2
  tag scope: e4=global
  wires:
  Subsystem1/1(e_d41) -> Equation (9)/1(e_d41)
  Equation (38)/1(alpha_pi) -> alpha_pi/1
  [e_dij_4_dot] -> Equation (38)/10(e_dij_dot)
  [pd4_dot] -> Equation (38)/7(pd_dot)
  MATLAB Function1/1(Ei) -> Ei/1, Equation (38)/5(Ei)
  [eij_4] -> MATLAB Function1/5(eij)
  Equation (15)/1(eta_e4) -> MATLAB Function1/2(eta_ei), Equation (38)/3(eta_ei)
  MATLAB Function/2(eta_eij) -> Equation (38)/6(eta_eij), MATLAB Function1/7(eta_eij)
  Equation (15)/2(d_eta_d_dei) -> MATLAB Function1/3(d_eta_d_dei), Equation (38)/4(d_eta_d_dei)
  Subsystem1/2(e_d42) -> Equation (9)/2(e_d42)
  MATLAB Function/1(d_eij) -> Equation (38)/12(d_eij)
  Subsystem/1(e41) -> Equation (10)/1(e41)
  Subsystem/3(e43) -> Equation (10)/3(e43)
  Clock1/1 -> MATLAB Function/2(t)
  MATLAB Function/3(d_eta_d_deij) -> Equation (38)/13(d_eta_d_deij), MATLAB Function1/8(d_eta_d_eij)
  [e_dij_4] -> Equation (38)/9(e_dij)
  p_d4/1 -> Add/2
  Clock/1 -> Equation (15)/2(t)
  Equation (9)/1(vij) -> Equation (38)/11(vij), MATLAB Function/3(vij)
  Equation (8)/1(dei) -> MATLAB Function1/1(dei), Equation (38)/2(dei), Equation (15)/1(dei)
  Subsystem/2(e42) -> Equation (10)/2(e42)
  [p4] -> Add/1
  Add/1 -> MATLAB Function1/4(ei), [e4], Equation (38)/1(ei), Equation (8)/1(ei)  "ei"
  Clock2/1 -> Equation (38)/8(t)
  Subsystem1/3(e_d43) -> Equation (9)/3(e_d43)
  Equation (10)/1(dij) -> MATLAB Function/1(dij), MATLAB Function1/6(d_ij)

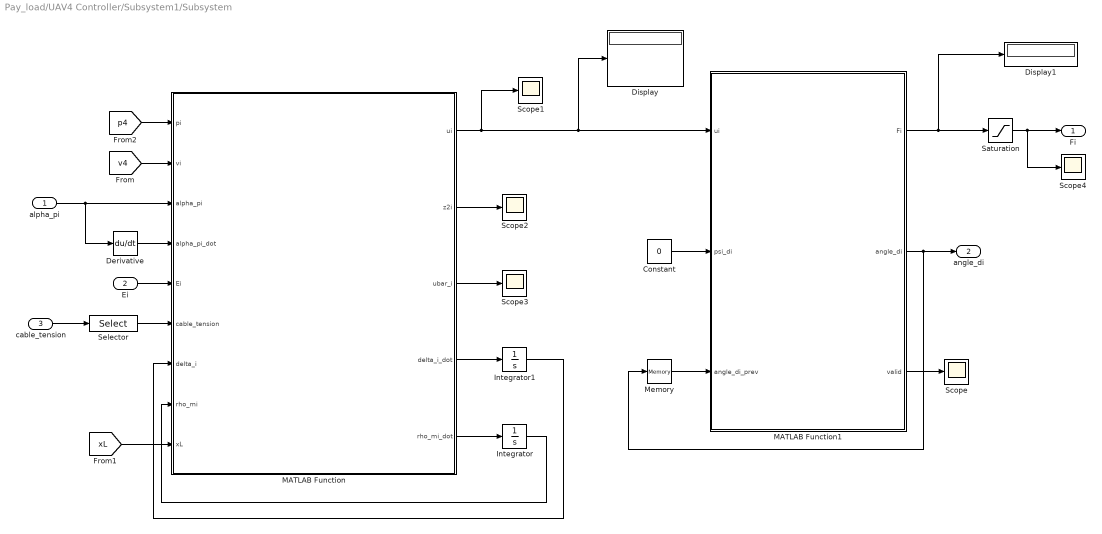
== system Pay_load/UAV4 Controller/Subsystem1/Subsystem ==
  alpha_pi : Inport
  Ei : Inport  Port=2
  cable_tension : Inport  Port=3
  Constant : Constant  Value=0
  Derivative : Derivative
  Display : Display
  Display1 : Display
  Integrator : Integrator  InitialCondition=1
  Integrator1 : Integrator
  MATLAB Function : MATLAB Function  TreatAsAtomicUnit=on  mask{ri=r4, m=m4}
      mask prompts: ri "Joint Vector"; m "UAV's Mass"
  MATLAB Function1 : MATLAB Function  TreatAsAtomicUnit=on
  Memory : Memory
  Saturation : Saturate  UpperLimit=75  LowerLimit=0
  Scope{,1..4} (5 alike) : Scope
      Scope settings: ActiveDisplayYMinimum=-1  ActiveDisplayYMaximum=1
      Scope1 settings: ActiveDisplayYMinimum=-3904.7073204545968  ActiveDisplayYMaximum=15673.723766073857  DataLoggingVariableName=ScopeData6
      Scope2 settings: ActiveDisplayYMinimum=-1  ActiveDisplayYMaximum=1  DataLoggingVariableName=ScopeData7
      Scope3 settings: ActiveDisplayYMinimum=-1  ActiveDisplayYMaximum=1  DataLoggingVariableName=ScopeData8
      Scope4 settings: ActiveDisplayYMinimum=-1  ActiveDisplayYMaximum=1  DataLoggingVariableName=ScopeData9
  Selector : Selector  InputPortWidth=12  IndexOptions=Index vector (dialog)  Indices=[10:12]  OutputSizes=1
  Fi : Outport
  angle_di : Outport  Port=2
  wires:
  [v4] -> MATLAB Function/2(vi)
  alpha_pi/1 -> Derivative/1, MATLAB Function/3(alpha_pi)
  Ei/1 -> MATLAB Function/5(Ei)
  Derivative/1 -> MATLAB Function/4(alpha_pi_dot)
  MATLAB Function/5(rho_mi_dot) -> Integrator/1
  MATLAB Function/4(delta_i_dot) -> Integrator1/1
  Integrator1/1 -> MATLAB Function/7(delta_i)
  Integrator/1 -> MATLAB Function/8(rho_mi)
  cable_tension/1 -> Selector/1
  Selector/1 -> MATLAB Function/6(cable_tension)
  [xL] -> MATLAB Function/9(xL)
  [p4] -> MATLAB Function/1(pi)
  MATLAB Function/1(ui) -> Scope1/1, Display/1, MATLAB Function1/1(ui)
  Constant/1 -> MATLAB Function1/2(psi_di)
  Memory/1 -> MATLAB Function1/3(angle_di_prev)
  MATLAB Function1/2(angle_di) -> angle_di/1, Memory/1
  MATLAB Function1/3(valid) -> Scope/1
  MATLAB Function1/1(Fi) -> Display1/1, Saturation/1
  Saturation/1 -> Scope4/1, Fi/1
  MATLAB Function/2(z2i) -> Scope2/1
  MATLAB Function/3(ubar_i) -> Scope3/1

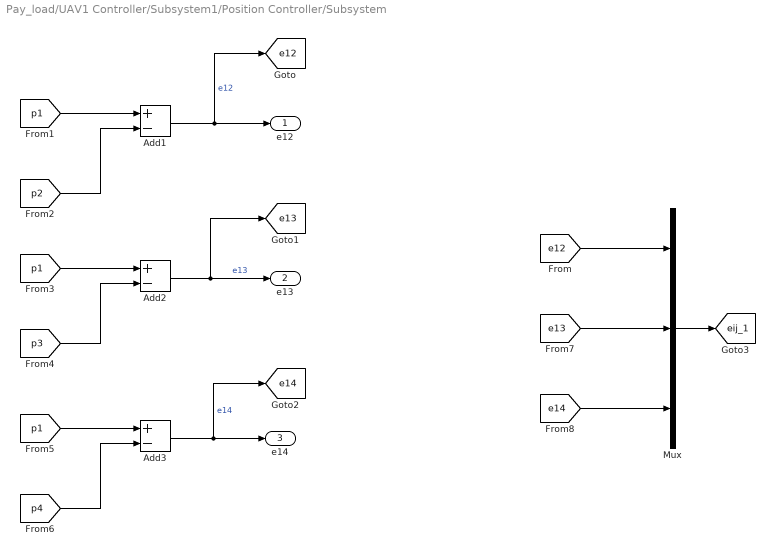
== system Pay_load/UAV1 Controller/Subsystem1/Position Controller/Subsystem ==
  Add1 : Sum  Inputs=+-
  Add2 : Sum  Inputs=+-
  Add3 : Sum  Inputs=+-
  Mux : Mux  Inputs=3
  e12 : Outport
  e13 : Outport  Port=2
  e14 : Outport  Port=3
  tag scope: e12=global, e13=global, e14=global, eij_1=global
  wires:
  [p4] -> Add3/2
  [p1] -> Add2/1
  Add2/1 -> [e13], e13/1  "e13"
  Add1/1 -> [e12], e12/1  "e12"
  Add3/1 -> [e14], e14/1  "e14"
  [p1] -> Add3/1
  [p3] -> Add2/2
  [p2] -> Add1/2
  [p1] -> Add1/1
  [e12] -> Mux/1
  [e13] -> Mux/2
  [e14] -> Mux/3
  Mux/1 -> [eij_1]

== system Pay_load/UAV1 Controller/Subsystem1/Position Controller/Subsystem1 ==
  Add4 : Sum  Inputs=+-
  Add5 : Sum  Inputs=+-
  Add6 : Sum  Inputs=+-
  Derivative : Derivative
  Mux : Mux  Inputs=3
  Scope : Scope
      settings: ActiveDisplayYMinimum=-1  ActiveDisplayYMaximum=1  DataLoggingVariableName=ScopeData14
  e_d12 : Outport
  e_d13 : Outport  Port=2
  e_d14 : Outport  Port=3
  tag scope: e_dij_1=global, e_dij_1_dot=global
  wires:
  [p_d1] -> Add6/1
  Add5/1 -> Mux/2, e_d13/1  "e_d13"
  [p_d1] -> Add4/1
  [p_d4] -> Add6/2
  [p_d2] -> Add4/2
  Add6/1 -> Mux/3, e_d14/1  "e_d14"
  [p_d3] -> Add5/2
  [p_d1] -> Add5/1
  Add4/1 -> Mux/1, e_d12/1  "e_d12"
  Mux/1 -> Derivative/1, [e_dij_1]
  Derivative/1 -> Scope/1, [e_dij_1_dot]

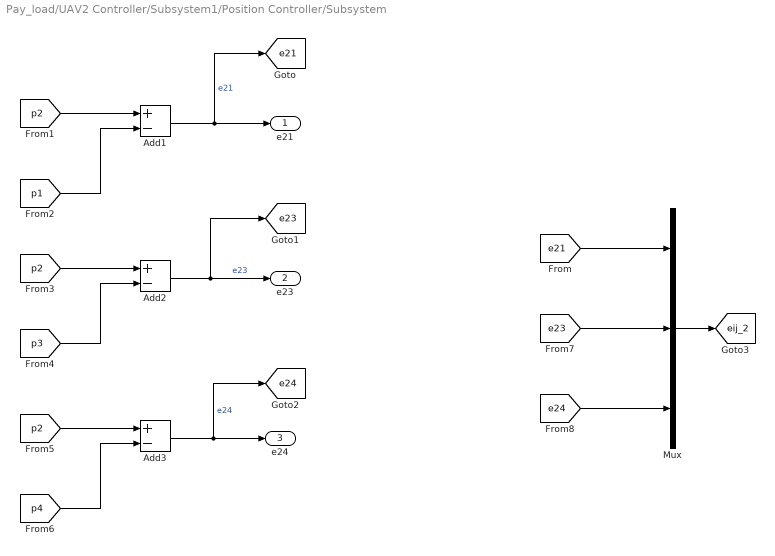
== system Pay_load/UAV2 Controller/Subsystem1/Position Controller/Subsystem ==
  Add1 : Sum  Inputs=+-
  Add2 : Sum  Inputs=+-
  Add3 : Sum  Inputs=+-
  Mux : Mux  Inputs=3
  e21 : Outport
  e23 : Outport  Port=2
  e24 : Outport  Port=3
  tag scope: e21=global, e23=global, e24=global, eij_2=global
  wires:
  [p4] -> Add3/2
  [p2] -> Add2/1
  Add2/1 -> [e23], e23/1  "e23"
  Add1/1 -> [e21], e21/1  "e21"
  Add3/1 -> [e24], e24/1  "e24"
  [p2] -> Add3/1
  [p3] -> Add2/2
  [p1] -> Add1/2
  [p2] -> Add1/1
  [e21] -> Mux/1
  [e23] -> Mux/2
  [e24] -> Mux/3
  Mux/1 -> [eij_2]

== system Pay_load/UAV2 Controller/Subsystem1/Position Controller/Subsystem1 ==
  Add4 : Sum  Inputs=+-
  Add5 : Sum  Inputs=+-
  Add6 : Sum  Inputs=+-
  Derivative : Derivative
  Mux : Mux  Inputs=3
  e_d21 : Outport
  e_d23 : Outport  Port=2
  e_d24 : Outport  Port=3
  tag scope: e_dij_2=global, e_dij_2_dot=global
  wires:
  [p_d2] -> Add6/1
  Add5/1 -> Mux/2, e_d23/1  "e_d23"
  [p_d2] -> Add4/1
  [p_d4] -> Add6/2
  [p_d1] -> Add4/2
  Add6/1 -> Mux/3, e_d24/1  "e_d24"
  [p_d3] -> Add5/2
  [p_d2] -> Add5/1
  Add4/1 -> Mux/1, e_d21/1  "e_d21"
  Mux/1 -> Derivative/1, [e_dij_2]
  Derivative/1 -> [e_dij_2_dot]

== system Pay_load/UAV3 Controller/Subsystem1/Position Controller/Subsystem ==
  Add1 : Sum  Inputs=+-
  Add2 : Sum  Inputs=+-
  Add3 : Sum  Inputs=+-
  Mux : Mux  Inputs=3
  e31 : Outport
  e32 : Outport  Port=2
  e34 : Outport  Port=3
  tag scope: e31=global, e32=global, e34=global, eij_3=global
  wires:
  [p4] -> Add3/2
  [p3] -> Add2/1
  Add2/1 -> [e32], e32/1  "e13"
  Add1/1 -> [e31], e31/1  "e12"
  Add3/1 -> [e34], e34/1  "e14"
  [p3] -> Add3/1
  [p2] -> Add2/2
  [p1] -> Add1/2
  [p3] -> Add1/1
  [e31] -> Mux/1
  [e32] -> Mux/2
  [e34] -> Mux/3
  Mux/1 -> [eij_3]

== system Pay_load/UAV3 Controller/Subsystem1/Position Controller/Subsystem1 ==
  Add4 : Sum  Inputs=+-
  Add5 : Sum  Inputs=+-
  Add6 : Sum  Inputs=+-
  Derivative : Derivative
  Mux : Mux  Inputs=3
  e_d31 : Outport
  e_d32 : Outport  Port=2
  e_d34 : Outport  Port=3
  tag scope: e_dij_3=global, e_dij_3_dot=global
  wires:
  [p_d3] -> Add6/1
  Add5/1 -> Mux/2, e_d32/1  "e_d32"
  [p_d3] -> Add4/1
  [p_d4] -> Add6/2
  [p_d1] -> Add4/2
  Add6/1 -> Mux/3, e_d34/1  "e_d34"
  [p_d2] -> Add5/2
  [p_d3] -> Add5/1
  Add4/1 -> Mux/1, e_d31/1  "e_d31"
  Mux/1 -> Derivative/1, [e_dij_3]
  Derivative/1 -> [e_dij_3_dot]

== system Pay_load/UAV4 Controller/Subsystem1/Position Controller/Subsystem ==
  Add1 : Sum  Inputs=+-
  Add2 : Sum  Inputs=+-
  Add3 : Sum  Inputs=+-
  Mux : Mux  Inputs=3
  e41 : Outport
  e42 : Outport  Port=2
  e43 : Outport  Port=3
  tag scope: e41=global, e42=global, e43=global, eij_4=global
  wires:
  [p3] -> Add3/2
  [p4] -> Add2/1
  Add2/1 -> [e42], e42/1  "e42"
  Add1/1 -> [e41], e41/1  "e41"
  Add3/1 -> [e43], e43/1  "e43"
  [p4] -> Add3/1
  [p2] -> Add2/2
  [p1] -> Add1/2
  [p4] -> Add1/1
  [e41] -> Mux/1
  [e42] -> Mux/2
  [e43] -> Mux/3
  Mux/1 -> [eij_4]

== system Pay_load/UAV4 Controller/Subsystem1/Position Controller/Subsystem1 ==
  Add4 : Sum  Inputs=+-
  Add5 : Sum  Inputs=+-
  Add6 : Sum  Inputs=+-
  Derivative : Derivative
  Mux : Mux  Inputs=3
  e_d41 : Outport
  e_d42 : Outport  Port=2
  e_d43 : Outport  Port=3
  tag scope: e_dij_4=global, e_dij_4_dot=global
  wires:
  [p_d4] -> Add6/1
  Add5/1 -> Mux/2, e_d42/1  "e_d42"
  [p_d4] -> Add4/1
  [p_d3] -> Add6/2
  [p_d1] -> Add4/2
  Add6/1 -> Mux/3, e_d43/1  "e_d43"
  [p_d2] -> Add5/2
  [p_d4] -> Add5/1
  Add4/1 -> Mux/1, e_d41/1  "e_d41"
  Mux/1 -> Derivative/1, [e_dij_4]
  Derivative/1 -> [e_dij_4_dot]

== matlab function Pay_load/PayLoad Controller/Adaptive law (22) ==
  data: z2L input; sigma_1L_dot output; sigma_1L input
function sigma_1L_dot = fcn(z2L, sigma_1L)

    n_delta1L = 0.25; epsilon_L = 0.1; gamma_delta1L = 0.1;

    sigma_1L_dot = 0;

    sigma_1L_dot = n_delta1L*(norm(z2L)^2/sqrt(norm(z2L)^2 + epsilon_L^2)) - gamma_delta1L*sigma_1L;

end

== matlab function Pay_load/PayLoad Controller/Equation (21) ==
  data: eta_eL input; deri input; EL input; alpha_pL_dot input; z2L input; Fdl output; sigma_1L input; mL parameter
function Fdl = fcn(eta_eL, deri, EL, alpha_pL_dot, z2L, sigma_1L, mL)

    K2L = 3.55; epsilon_L = 0.1;

    g = 9.81; 
    
    ez = [0, 0, 1]';

    Fdl = mL*g*ez - mL*alpha_pL_dot + K2L*z2L + eta_eL*deri*EL + sigma_1L*(z2L/sqrt(norm(z2L)^2 + epsilon_L^2));

end

== matlab function Pay_load/PayLoad Controller/Equation (25) ==
  data: z3L output; Gamma_L output; Psi_L output; angle_L input; alpha_angle_L output; angle_dL input; angle_dL_dot input
function [z3L, Gamma_L, Psi_L, alpha_angle_L]= fcn(angle_L, angle_dL, angle_dL_dot)

    K3L = 2.35;

    phi_L = angle_L(1); theta_L = angle_L(2); psi_L = angle_L(3);

    Gamma_L = [1, sin(phi_L)*tan(theta_L), cos(phi_L)*tan(theta_L);
                0, cos(phi_L), -sin(phi_L);
                0, sin(phi_L)/cos(theta_L), cos(phi_L)/cos(theta_L)];

    Psi_L = Gamma_L \ eye(3);

    z3L = angle_L - angle_dL;

    alpha_angle_L = -K3L*z3L + angle_dL_dot;

end

== matlab function Pay_load/PayLoad Controller/Equation (27) ==
  data: Gamma_L input; z3L input; sq_L input; z4L input; M_dL output; rho_jL input; eta_L input; delta_2L input; muy_L output
function [M_dL, muy_L]= fcn(Gamma_L, z3L, sq_L, z4L, rho_jL, eta_L, delta_2L)

    epsilon_L = 0.1; K4L = 2.35;

    M_dL = zeros(3,1);


    %% Equation (28)
    muy_L = K4L*Gamma_L'*z4L + Gamma_L'*z3L + eta_L*(Gamma_L'*z4L*sq_L^2)/sqrt(norm(z4L)^2 * sq_L^2 + epsilon_L^2) + delta_2L*Gamma_L'*z4L/sqrt(norm(z4L)^2 + epsilon_L^2);

    Psi_L = Gamma_L \ eye(3);


    %% Equation (27)
    M_dL = (Psi_L*z4L*norm(muy_L)^2*(rho_jL*rho_jL'))/(sqrt(norm(Psi_L*z4L)^2 * norm(muy_L)^2 * (rho_jL*rho_jL') + epsilon_L^2));

end

== matlab function Pay_load/PayLoad Controller/Subsystem/Adaptive Law (eq. 29) ==
  data: z4L input; rho_jL input; rho_jL_dot output; Gamma_L input; muy_L input
function rho_jL_dot = fcn(z4L, rho_jL, Gamma_L, muy_L)

    n_rhoJL = 0.25; sigma_rhoJL = 0.1; 

    Psi_L = Gamma_L \ eye(3);

    rho_jL_dot = n_rhoJL*z4L'*Psi_L'*muy_L - sigma_rhoJL*rho_jL;

end

== matlab function Pay_load/PayLoad Controller/Subsystem/Adaptive Law (eq. 30) ==
  data: z4L input; eta_L input; eta_L_dot output; sq_L input
function eta_L_dot = fcn(z4L, eta_L, sq_L)

    n_etaL = 0.25; sigma_etaL = 0.1; epsilon_L = 0.1;

    eta_L_dot = n_etaL*norm(z4L)^2*sq_L^2/sqrt(norm(z4L)^2*sq_L^2 + epsilon_L^2) - sigma_etaL*eta_L;

end
